simulink model "Shaddad_BMS"  (R2026b)
undefined symbols (not defined in the file): CAN, FD, P, Ts
libraries: simulink x39, stm32blockslib x12, BatteryProtection x7, dspstat3 x7, BatteryEstimators x4, BatteryCurrentManagement x3, eeGeneralControl x2, BatteryBalancing x1, BatterySoeEstimators x1, BatteryPowerEstimators x1, BatteryThermalManagement x1, svdutilitieslib x1
(part 1 of 2)
settings Model: Creator=aomar  LastModifiedBy=aomar

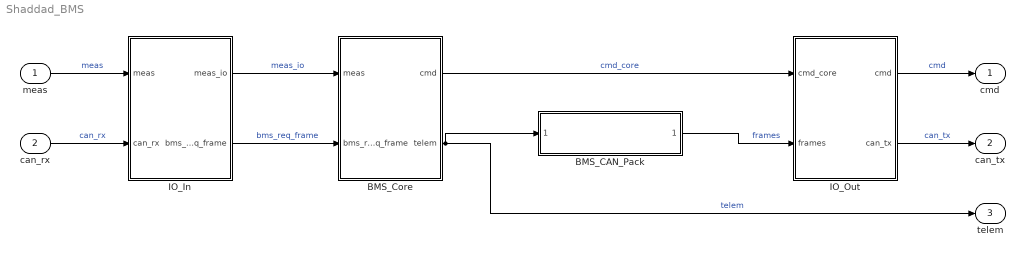
== system Shaddad_BMS ==
  meas : Inport  OutDataTypeStr=Bus: Bus_BMS_Meas  SampleTime=Ts.bms_fast  BusOutputAsStruct=on
  can_rx : Inport  Port=2  OutDataTypeStr=Bus: Bus_Can1_McuSlow  SampleTime=Ts.can_slow  BusOutputAsStruct=on
  BMS_CAN_Pack : Subsystem  ReferencedSubsystem=bms_can_pack
  BMS_Core : Subsystem  TreatAsAtomicUnit=on
  IO_In : Subsystem  Variant=on
  IO_Out : Subsystem  Variant=on
  cmd : Outport  OutDataTypeStr=Bus: Bus_BMS_Cmd  SampleTime=Ts.bms_fast  BusOutputAsStruct=on
  can_tx : Outport  Port=2  OutDataTypeStr=Bus: Bus_Can1_Bms  SampleTime=Ts.hk  BusOutputAsStruct=on
  telem : Outport  Port=3  OutDataTypeStr=Bus: Bus_BMS_Telemetry  SampleTime=Ts.hk  BusOutputAsStruct=on
  wires:
  meas/1 -> IO_In/1(meas)  "meas"
  can_rx/1 -> IO_In/2(can_rx)  "can_rx"
  IO_In/1(meas_io) -> BMS_Core/1(meas)  "meas_io"
  IO_In/2(bms_req_frame) -> BMS_Core/2(bms_req_frame)  "bms_req_frame"
  BMS_Core/1(cmd) -> IO_Out/1(cmd_core)  "cmd_core"
  BMS_Core/2(telem) -> telem/1, BMS_CAN_Pack/1  "telem"
  BMS_CAN_Pack/1 -> IO_Out/2(frames)  "frames"
  IO_Out/1(cmd) -> cmd/1  "cmd"
  IO_Out/2(can_tx) -> can_tx/1  "can_tx"

== system Shaddad_BMS/BMS_Core ==
  meas : Inport  OutDataTypeStr=Bus: Bus_BMS_Meas
  bms_req_frame : Inport  Port=2  OutDataTypeStr=Bus: Bus_CanFrame8
  BMS_REQ_Decode : Subsystem  ReferencedSubsystem=bmsreq_can_unpack
  Balancing : Subsystem  Description=Balancing (1 s): E16 Passive Cell Balancing (10 mV threshold, 3 mV hysteresis) enabled when (CHARGING or REST) and V_max > 3.40 V; E6 cell contact monitoring (gated off by P.power.bms.contact_enable).
  ChargeCtrl : Subsystem  Description=Charge control (0.1 s): E15 CC-CV on V_max (CV 3.55 V), request = min(CC-CV, I_chg_lim, 100 A) while CHARGING; E21 charge complete (V_max >= 3.545 V and I < 10 A for 60 s).
  CmdOut : Subsystem  Description=Bus_BMS_Cmd assembly; balancing gated at 10 ms ((CHARGING (K4 request) or |I| < I_rest) and V_max > 3.40 V); Unit Delay (0.01 s) = BMS output stage and the plant -> BMS -> plant loop breaker (E24).
  Estimation : Subsystem  Description=Estimation (0.1 s; capacity LS at 1 s): E7 SOC EKF x16 (variable capacity, D48; cell voltages corrected by the R0 ageing ratio R0a_* learned at current steps), E8 coulomb counting, E10 capacity (rate limit AH_rate_lim, bounds AH_bounds), E11 SOH, E12 SOE (EnergyCapacity = CellAH x 51.2 V), E9 power capability, E20 moving average of P_pack (P_avg_window samples at 1 s = 600 s), E_remaining = E_cap x max(SOC_pack - 0.10, 0), Runtime = 3600 E_remaining / max(P_avg, 200 W).
  FaultWord : Subsystem  Description=Fault_Word = latched protection bits | b6 PRECHARGE_FAIL | b7 K1_WELD | b16 SAFETY_OPEN | b20 MCU_CMD_TIMEOUT (b17-19 LV: no rail measurement at the BMS); Warning_Word b0-b7; Fault_Level 3/2/1/0 from P.power.bms.fault masks.
  Limits : Subsystem  Description=Current limits (0.01 s): E13 / E14 (MinMax inputs, temperature tables, voltage headroom), E22 SOC taper on SOC_min, peak / charge maxima. Outputs are magnitudes (A).
  Meas : Subsystem  Description=Measurement conditioning (0.01 s): min/max with index (dspstat3), mean, [min;max] pairs, I_lib = -I_pack (batt_sl_lib + = charge), P_pack.
  ModeManager : Subsystem  Description=Mode manager (0.01 s): MATLAB Function BMS_ModeManager (spec 4.1 transition table, enum BmsContactorState, after() tick counters, P.power.bms.chart), Safety_OK input = meas.Safety_HV_OK (stop-category-1 coil supply), MCU command timeout (BMS_REQ alive frozen 0.5 s -> HV_Enable_Req false, Fault_Word b20), Fault_Reset_Req rising edge for the protection latch.
  Protection : Subsystem  Description=Protection (0.01 s): E1 critical / E2 warning voltage monitoring, E3 overcurrent, E4 temperature, E5 fault qualification (fuses, charger OVP), E6 gate; fault bits latched until a Fault_Reset_Req rising edge with the symptom gone (library DisqualTime 0 would never clear, so P.power.bms.disqual is used).
  RT_req : RateTransition  OutPortSampleTime=Ts.bms_fast
  RT_req_valid : RateTransition  OutPortSampleTime=Ts.bms_fast
  Telemetry : Subsystem  Description=Telemetry (0.1 s): Bus_BMS_Telemetry with AliveCounter (+1 per 0.1 s), fault / warning words, contactor state, CVL / DVL.
  Thermal : Subsystem  Description=Fan control (0.1 s): E17 Battery Coolant Control ON-OFF 40 / 35 C on [T_min; T_max], AND T_max > T_amb - 1 K, OR T_max > 50 C.
  cmd : Outport  OutDataTypeStr=Bus: Bus_BMS_Cmd
  telem : Outport  Port=2  OutDataTypeStr=Bus: Bus_BMS_Telemetry
  wires:
  meas/1 -> Meas/1(meas)  "meas"
  bms_req_frame/1 -> BMS_REQ_Decode/1  "bms_req_frame"
  Meas/1(m) -> Limits/1(m), Thermal/1(m), ChargeCtrl/1(m), Protection/1(m), Telemetry/1(m), FaultWord/1(m), Balancing/1(m), Estimation/1(m), CmdOut/1(m), ModeManager/1(m)  "m"
  BMS_REQ_Decode/1 -> RT_req/1  "bms_req"
  BMS_REQ_Decode/2 -> RT_req_valid/1  "bms_req_valid"
  RT_req/1 -> ModeManager/2(req)  "req"
  RT_req_valid/1 -> ModeManager/3(req_valid)  "req_valid"
  Estimation/1(est) -> Limits/2(est), Telemetry/3(est), FaultWord/4(est)  "est"
  Thermal/1(Fan_Cmd) -> CmdOut/4(Fan_Cmd), FaultWord/6(Fan_Cmd), Telemetry/7(Fan_Cmd)  "Fan_Cmd"
  ModeManager/1(mode) -> CmdOut/2(mode), ChargeCtrl/2(mode), Balancing/2(mode), FaultWord/3(mode), Protection/2(mode), Telemetry/2(mode)  "mode"
  Limits/1(I_dis_lim) -> Protection/4(I_dis_lim), Telemetry/5(I_dis_lim)  "I_dis_lim"
  Limits/2(I_chg_lim) -> Protection/3(I_chg_lim), ChargeCtrl/3(I_chg_lim), Telemetry/6(I_chg_lim)  "I_chg_lim"
  Limits/3(derate) -> FaultWord/5(derate)  "derate"
  Balancing/1(Bal_Cmd) -> CmdOut/3(Bal_Cmd)  "Bal_Cmd"
  Balancing/2(Balancing_Active) -> Telemetry/9(Balancing_Active)  "Balancing_Active"
  Balancing/3(contact_err) -> Protection/5(contact_err)  "contact_err"
  ChargeCtrl/1(I_req) -> CmdOut/5(I_req)  "I_req"
  ChargeCtrl/2(ChargeComplete) -> ModeManager/5(ChargeComplete)  "ChargeComplete"
  CmdOut/1(cmd) -> cmd/1  "cmd"
  CmdOut/2(Bal_Cmd_out) -> Telemetry/8(Bal_Cmd)  "Bal_Cmd_out"
  Protection/1(prot) -> FaultWord/2(prot), ModeManager/4(prot)  "prot"
  FaultWord/1(fw) -> Telemetry/4(fw)  "fw"
  Telemetry/1(telem) -> telem/1  "telem"

== system Shaddad_BMS/IO_In ==
  note: 1) Add Subsystem or Model blocks as valid variant choices.
      | 2) You cannot connect blocks at this level. At simulation, connectivity is automatically
      | determined, based on the active variant and port name matching.
  meas : Inport
  can_rx : Inport  Port=2
  HW : Subsystem  Description=HW IO_In (VC_TARGET == 1): SPI AFE + afe_decode (block-based register decode), ADC1 6 channels, GPIO aux contacts (Digital Port Read GPIOC[4:11], one boolean per pin -> Demux), FDCAN1 read of 0x3D0 (Data [64x1] -> bytes 1:8, Length, Id; valid = Id == BMS_REQ). Peripheral settings / pin maps are configured by T17 (CubeMX, build_targets('peripherals')).  VariantControl=VC_TARGET == 1
  SIM : Subsystem  VariantControl=VC_TARGET == 0
  meas_io : Outport
  bms_req_frame : Outport  Port=2

== system Shaddad_BMS/IO_Out ==
  note: 1) Add Subsystem or Model blocks as valid variant choices.
      | 2) You cannot connect blocks at this level. At simulation, connectivity is automatically
      | determined, based on the active variant and port name matching.
  cmd_core : Inport
  frames : Inport  Port=2
  HW : Subsystem  Description=HW IO_Out (VC_TARGET == 1): contactor / charger / balancing GPIO, FDCAN1 raw-data transmit of the 7 BMS frames (inputs Data, Length, Id; Digital Port Write GPIOB[4 5 6 7 10] = K1 K2 K4 CHARGER_EN BAL_EN = OR(Bal_Cmd); pin maps from shaddad_g474.ioc, T17). Root outputs keep the SIM buses.  VariantControl=VC_TARGET == 1
  SIM : Subsystem  VariantControl=VC_TARGET == 0
  cmd : Outport
  can_tx : Outport  Port=2

== system Shaddad_BMS/BMS_Core/Balancing ==
  m_V_cell : Inport  PortName=m  Element=V_cell
  m_V_max : Inport  PortName=m  Element=V_max
  m_I_dis : Inport  PortName=m  Element=I_dis
  mode_Charging_Active : Inport  Port=2  PortName=mode  Element=Charging_Active
  Bal_enable : Logic  AllPortsSameDT=off  OutDataTypeStr=boolean
  Chg_or_rest : Logic  Operator=OR  AllPortsSameDT=off  OutDataTypeStr=boolean
  E16_Passive_balancing : BatteryBalancing/Passive Cell Balancing  Threshold=single(P.power.bms.bal.Threshold)  HysteresisBand=single(P.power.bms.bal.Hyst)  Td_on=P.power.bms.bal.Td_on  Td_off=P.power.bms.bal.Td_off  Ts=Ts.bms_bal  dataType=boolean
      settings: LibrarySourceBlock=batt_sl_lib/Cell Balancing/Passive Cell Balancing
  E6_Cell_contact : BatteryProtection/Battery Cell Contact Monitoring  Td=10  VoltageChangeDetectionThreshold=single(5e-4)  VoltageChangePar=single(0.02)  CumulativeErrorThreshold=single(1e-4)  QualTime=20  DisqualTime=0  Ts=Ts.bms_bal  DataType=single
      settings: LibrarySourceBlock=|
      | batt_sl_lib/Protection/Battery Cell Contact
      | Monitoring
  E6_any : Logic  Operator=OR  Inputs=1  AllPortsSameDT=off  OutDataTypeStr=boolean
  E6_symptom : Terminator
  I_abs : Abs  SaturateOnIntegerOverflow=off
  RT_I_dis : RateTransition  OutPortSampleTime=Ts.bms_bal
  RT_V_cell : RateTransition  OutPortSampleTime=Ts.bms_bal
  RT_V_max : RateTransition  OutPortSampleTime=Ts.bms_bal
  RT_active : RateTransition  OutPortSampleTime=Ts.bms_bal
  RT_contact : RateTransition  OutPortSampleTime=Ts.bms_fast
  Rest : simulink/Logic and Bit Operations/Compare To Constant  relop=<  const=single(P.power.bms.I_rest)  OutDataTypeStr=boolean
  Top : simulink/Logic and Bit Operations/Compare To Constant  relop=>  const=single(P.power.bms.V_bal_enable)  OutDataTypeStr=boolean
  Bal_Cmd : Outport
  Balancing_Active : Outport  Port=2
  contact_err : Outport  Port=3
  wires:
  m_I_dis/1 -> RT_I_dis/1  "I_dis"
  m_V_cell/1 -> RT_V_cell/1  "V_cell"
  RT_I_dis/1 -> I_abs/1  "RT_I_dis"
  RT_V_cell/1 -> E16_Passive_balancing/1, E6_Cell_contact/1  "RT_V_cell"
  I_abs/1 -> Rest/1  "I_abs"
  E6_Cell_contact/1 -> E6_any/1  "E6_Cell_contact_1"
  E6_Cell_contact/2 -> E6_symptom/1  "E6_Cell_contact_2"
  mode_Charging_Active/1 -> RT_active/1  "Charging_Active"
  m_V_max/1 -> RT_V_max/1  "V_max"
  Rest/1 -> Chg_or_rest/2  "Rest"
  RT_active/1 -> Chg_or_rest/1  "RT_active"
  RT_V_max/1 -> Top/1  "RT_V_max"
  Chg_or_rest/1 -> Bal_enable/1  "Chg_or_rest"
  Top/1 -> Bal_enable/2  "Top"
  Bal_enable/1 -> E16_Passive_balancing/2  "bal_enable"
  E6_any/1 -> RT_contact/1  "E6_any"
  RT_contact/1 -> contact_err/1  "contact_err"
  E16_Passive_balancing/1 -> Bal_Cmd/1  "Bal_Cmd"
  E16_Passive_balancing/2 -> Balancing_Active/1  "Balancing_Active"

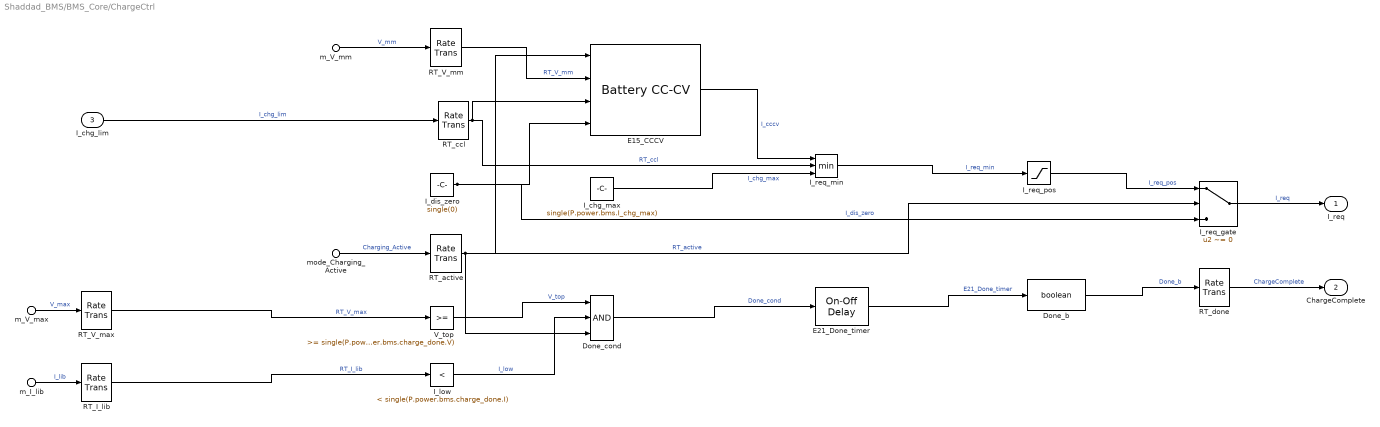
== system Shaddad_BMS/BMS_Core/ChargeCtrl ==
  m_V_mm : Inport  PortName=m  Element=V_mm
  m_V_max : Inport  PortName=m  Element=V_max
  m_I_lib : Inport  PortName=m  Element=I_lib
  mode_Charging_Active : Inport  Port=2  PortName=mode  Element=Charging_Active
  I_chg_lim : Inport  Port=3
  Done_b : DataTypeConversion  OutDataTypeStr=boolean  SaturateOnIntegerOverflow=off  RndMeth=Floor
  Done_cond : Logic  Inputs=3  AllPortsSameDT=off  OutDataTypeStr=boolean
  E15_CCCV : BatteryCurrentManagement/Battery CC-CV  MinMaxFlag=on  MaxCellVoltage=single(P.power.bms.V_cv)  Kp=single(P.power.bms.cccv.Kp)  Ki=single(P.power.bms.cccv.Ki)  Kaw=single(P.power.bms.cccv.Kaw)  Kt=single(P.power.bms.cccv.Kt)  Ts=Ts.bms_slow
      settings: LibrarySourceBlock=batt_sl_lib/Current Management/Battery CC-CV
  E21_Done_timer : eeGeneralControl/On-Off Delay  LabelModeActiveChoice=Discrete  Td_on=P.power.bms.charge_done.t  Td_off=0  IC=0  Ts=Ts.bms_slow
      settings: LibrarySourceBlock=ee_sl_lib/General Control/On-Off Delay
  I_chg_max : Constant  Value=single(P.power.bms.I_chg_max)  OutDataTypeStr=single  SampleTime=Ts.bms_slow
  I_dis_zero : Constant  Value=single(0)  OutDataTypeStr=single  SampleTime=Ts.bms_slow
  I_low : simulink/Logic and Bit Operations/Compare To Constant  relop=<  const=single(P.power.bms.charge_done.I)  OutDataTypeStr=boolean
  I_req_gate : Switch  Criteria=u2 ~= 0  SaturateOnIntegerOverflow=off  InputSameDT=off
  I_req_min : MinMax  Inputs=3
  I_req_pos : Saturate  UpperLimit=inf  LowerLimit=single(0)
  RT_I_lib : RateTransition  OutPortSampleTime=Ts.bms_slow
  RT_V_max : RateTransition  OutPortSampleTime=Ts.bms_slow
  RT_V_mm : RateTransition  OutPortSampleTime=Ts.bms_slow
  RT_active : RateTransition  OutPortSampleTime=Ts.bms_slow
  RT_ccl : RateTransition  OutPortSampleTime=Ts.bms_slow
  RT_done : RateTransition  OutPortSampleTime=Ts.bms_fast
  V_top : simulink/Logic and Bit Operations/Compare To Constant  relop=>=  const=single(P.power.bms.charge_done.V)  OutDataTypeStr=boolean
  I_req : Outport
  ChargeComplete : Outport  Port=2
  wires:
  m_V_max/1 -> RT_V_max/1  "V_max"
  m_I_lib/1 -> RT_I_lib/1  "I_lib"
  I_chg_lim/1 -> RT_ccl/1  "I_chg_lim"
  RT_V_max/1 -> V_top/1  "RT_V_max"
  RT_I_lib/1 -> I_low/1  "RT_I_lib"
  m_V_mm/1 -> RT_V_mm/1  "V_mm"
  mode_Charging_Active/1 -> RT_active/1  "Charging_Active"
  I_dis_zero/1 -> E15_CCCV/4, I_req_gate/3  "I_dis_zero"
  V_top/1 -> Done_cond/1  "V_top"
  I_low/1 -> Done_cond/2  "I_low"
  RT_V_mm/1 -> E15_CCCV/2  "RT_V_mm"
  RT_active/1 -> E15_CCCV/1, Done_cond/3, I_req_gate/2  "RT_active"
  RT_ccl/1 -> I_req_min/2, E15_CCCV/3  "RT_ccl"
  I_chg_max/1 -> I_req_min/3  "I_chg_max"
  Done_cond/1 -> E21_Done_timer/1  "Done_cond"
  E15_CCCV/1 -> I_req_min/1  "I_cccv"
  I_req_min/1 -> I_req_pos/1  "I_req_min"
  E21_Done_timer/1 -> Done_b/1  "E21_Done_timer"
  I_req_pos/1 -> I_req_gate/1  "I_req_pos"
  Done_b/1 -> RT_done/1  "Done_b"
  RT_done/1 -> ChargeComplete/1  "ChargeComplete"
  I_req_gate/1 -> I_req/1  "I_req"

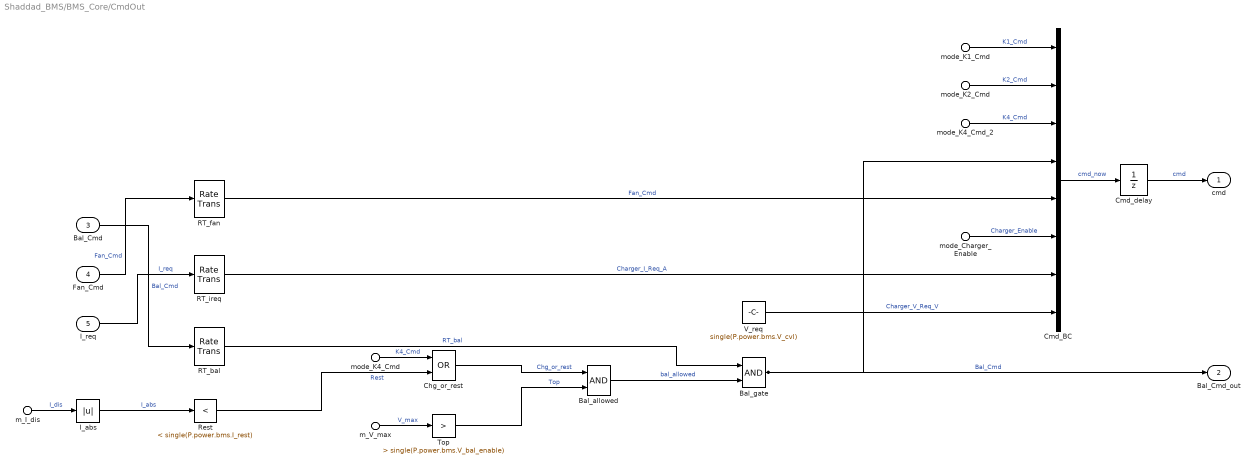
== system Shaddad_BMS/BMS_Core/CmdOut ==
  m_I_dis : Inport  PortName=m  Element=I_dis
  m_V_max : Inport  PortName=m  Element=V_max
  mode_K4_Cmd : Inport  Port=2  PortName=mode  Element=K4_Cmd
  mode_K4_Cmd_2 : Inport  Port=2  PortName=mode  Element=K4_Cmd
  mode_K1_Cmd : Inport  Port=2  PortName=mode  Element=K1_Cmd
  mode_K2_Cmd : Inport  Port=2  PortName=mode  Element=K2_Cmd
  mode_Charger_Enable : Inport  Port=2  PortName=mode  Element=Charger_Enable
  Bal_Cmd : Inport  Port=3
  Fan_Cmd : Inport  Port=4
  I_req : Inport  Port=5
  Bal_allowed : Logic  AllPortsSameDT=off  OutDataTypeStr=boolean
  Bal_gate : Logic  AllPortsSameDT=off  OutDataTypeStr=boolean
  Chg_or_rest : Logic  Operator=OR  AllPortsSameDT=off  OutDataTypeStr=boolean
  Cmd_BC : BusCreator  Inputs=8  OutDataTypeStr=Bus: Bus_BMS_Cmd  NonVirtualBus=on
      settings: InheritFromInputs=off
  Cmd_delay : UnitDelay  InitialCondition=P.ic.Bus_BMS_Cmd  SampleTime=Ts.bms_fast
  I_abs : Abs  SaturateOnIntegerOverflow=off
  RT_bal : RateTransition  OutPortSampleTime=Ts.bms_fast
  RT_fan : RateTransition  OutPortSampleTime=Ts.bms_fast
  RT_ireq : RateTransition  OutPortSampleTime=Ts.bms_fast
  Rest : simulink/Logic and Bit Operations/Compare To Constant  relop=<  const=single(P.power.bms.I_rest)  OutDataTypeStr=boolean
  Top : simulink/Logic and Bit Operations/Compare To Constant  relop=>  const=single(P.power.bms.V_bal_enable)  OutDataTypeStr=boolean
  V_req : Constant  Value=single(P.power.bms.V_cvl)  OutDataTypeStr=single  SampleTime=Ts.bms_fast
  cmd : Outport
  Bal_Cmd_out : Outport  Port=2
  wires:
  m_I_dis/1 -> I_abs/1  "I_dis"
  Bal_Cmd/1 -> RT_bal/1  "Bal_Cmd"
  Fan_Cmd/1 -> RT_fan/1  "Fan_Cmd"
  I_req/1 -> RT_ireq/1  "I_req"
  I_abs/1 -> Rest/1  "I_abs"
  Rest/1 -> Chg_or_rest/2  "Rest"
  RT_fan/1 -> Cmd_BC/5  "Fan_Cmd"
  RT_ireq/1 -> Cmd_BC/7  "Charger_I_Req_A"
  RT_bal/1 -> Bal_gate/1  "RT_bal"
  mode_K4_Cmd/1 -> Chg_or_rest/1  "K4_Cmd"
  m_V_max/1 -> Top/1  "V_max"
  Chg_or_rest/1 -> Bal_allowed/1  "Chg_or_rest"
  Top/1 -> Bal_allowed/2  "Top"
  Bal_allowed/1 -> Bal_gate/2  "bal_allowed"
  V_req/1 -> Cmd_BC/8  "Charger_V_Req_V"
  Bal_gate/1 -> Cmd_BC/4, Bal_Cmd_out/1  "Bal_Cmd"
  mode_K1_Cmd/1 -> Cmd_BC/1  "K1_Cmd"
  mode_K2_Cmd/1 -> Cmd_BC/2  "K2_Cmd"
  mode_K4_Cmd_2/1 -> Cmd_BC/3  "K4_Cmd"
  mode_Charger_Enable/1 -> Cmd_BC/6  "Charger_Enable"
  Cmd_BC/1 -> Cmd_delay/1  "cmd_now"
  Cmd_delay/1 -> cmd/1  "cmd"

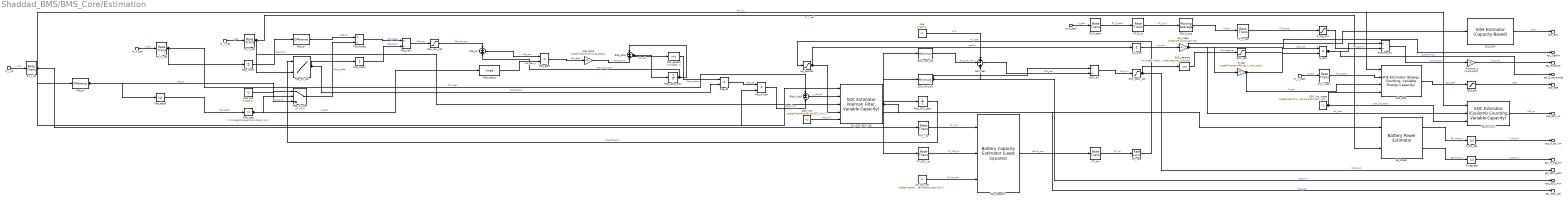
== system Shaddad_BMS/BMS_Core/Estimation ==
  m_I_lib : Inport  PortName=m  Element=I_lib
  m_V_cell : Inport  PortName=m  Element=V_cell
  m_T_cell : Inport  PortName=m  Element=T_cell
  m_V_pack : Inport  PortName=m  Element=V_pack
  m_P_pack : Inport  PortName=m  Element=P_pack
  AH_bounds : Saturate  UpperLimit=single(P.power.bms.est.AH_bounds(2))  LowerLimit=single(P.power.bms.est.AH_bounds(1))
  AH_init_vec : Constant  Value=single(P.power.bms.est.AH_init*ones(P.power.pack.Ns,1))  OutDataTypeStr=single  SampleTime=Ts.bms_bal
  AH_mean : Gain  Gain=single(1/P.power.pack.Ns)
  AH_rate : RateLimiter  RisingSlewLimit=single(P.power.bms.est.AH_rate_lim)  FallingSlewLimit=single(-P.power.bms.est.AH_rate_lim)  SampleTimeMode=inherited  InitialCondition=single(P.power.bms.est.AH_init)
  AH_sum : Sum  Inputs=+
  E10_Capacity : BatteryEstimators/Battery Capacity Estimator (Least Squares)  CurrentInputPartition=off  lsAlgorithm=Ordinary least squares  SocChangeThreshold=single(P.power.bms.cap_est.SocChangeThreshold)  gamma=single(P.power.bms.cap_est.gamma)  VarianceX=2e-4  VarianceY=5e-7  k=10  Ts=P.power.bms.cap_est.Ts  DataType=single
      settings: LibrarySourceBlock=|
      | batt_sl_lib/Estimators/Battery Capacity Estimator
      | (Least Squares)
  E11_SOH : BatteryEstimators/SOH Estimator (Capacity-Based)  AH_new=single(P.power.bms.soh.AH_new)  AH_eol=single(P.power.bms.soh.AH_eol)  DataType=single
      settings: LibrarySourceBlock=batt_sl_lib/Estimators/SOH Estimator (Capacity-Based)
  E12_SOE : BatterySoeEstimators/SOE Estimator (Energy Counting, Variable Energy Capacity)  CurrentInputPartition=off  Ts=Ts.bms_slow  DataType=single
      settings: LibrarySourceBlock=|
      | batt_sl_lib/Estimators/SOE Estimator (Energy Counting,
      | Variable Energy Capacity)
  E20_P_avg : dspstat3/Moving Average  Method=Sliding window  ForgettingFactorPort=off  SpecifyWindowLength=on  WindowLengthSource=Property  MaxWindowLength=20  WindowLength=P.power.bms.P_avg_window  OverlapLength=P.power.bms.P_avg_window - 1  AllowArbitraryInputLength=off  ForgettingFactor=0.9  SimulateUsing=Interpreted execution
  E7_SOC_EKF_x16 : BatteryEstimators/SOC Estimator (Kalman Filter, Variable Capacity)  CurrentInputPartition=off  filterType=Extended Kalman filter  alpha=1  beta=2  kappa=0  Q=single(P.power.bms.ekf.Q)  Q_2RC=|  R=single(P.power.bms.ekf.R)  P0=single(P.power.bms.ekf.P0)  P0_2RC=[1e-5 0 0; 0 1 0;0 0 1]  Ts=Ts.bms_slow  chargeDynamics=One time-constant dynamics  SOC_vec=single(P.power.group.SOC_vec)  T_vec=single(P.power.group.T_vec)  R0_mat=single(P.power.group.R0_mat)  R1_mat=single(P.power.group.R1_mat)  tau1_mat=single(P.power.group.tau1_mat)  R2_mat=[.0109, .0029, .0013; .0069, .0024, .0012; .0047, .0026, .0013; .0034, .0016, .001; .0033, .0023, .0014; .0033, .0018, .0011; .0028, .0017, .0011]  tau2_mat=[20, 36, 39; 31, 45, 39; 109, 105, 61; 36, 29, 26; 59, 77, 67; 40, 33, 29; 25, 39, 33]  V0_mat=single(P.power.group.V0_mat)  DataType=single
      | [1e-6 0 0;
      | 0 1e-6 0;0 0 1e-6]
      settings: LibrarySourceBlock=|
      | batt_sl_lib/Estimators/SOC Estimator
      | (Kalman Filter, Variable Capacity)
  E8_SOC_CC : BatteryEstimators/SOC Estimator (Coulomb Counting, Variable Capacity)  CurrentInputPartition=off  Ts=Ts.bms_slow  DataType=single
      settings: LibrarySourceBlock=|
      | batt_sl_lib/Estimators/SOC Estimator
      | (Coulomb Counting, Variable Capacity)
  E9_Power : BatteryPowerEstimators/Battery Power Estimator  SOC_vec=single(P.power.group.SOC_vec)  T_vec=single(P.power.group.T_vec)  V0_mat=single(P.power.group.V0_mat)  R0ChargingTimeHorizon=single(P.power.bms.pwr_est.R_10s)  R0DischargingTimeHorizon=single(P.power.bms.pwr_est.R_10s)  AH=single(P.power.group.AH)  Ns=P.power.pack.Ns  Np=1  ChargingEfficiency=single(P.power.bms.pwr_est.ChargingEfficiency)  vmin=single(P.power.bms.pwr_est.vmin)  vmax=single(P.power.bms.pwr_est.vmax)  SOCmin=single(P.power.bms.pwr_est.SOCmin)  SOCmax=single(P.power.bms.pwr_est.SOCmax)  imin=single(P.power.bms.pwr_est.imin)  imax=single(P.power.bms.pwr_est.imax)  Pmin=single(P.power.bms.pwr_est.Pmin)  Pmax=single(P.power.bms.pwr_est.Pmax)  TimeHorizon=single(P.power.bms.pwr_est.TimeHorizon)  DataType=single
      settings: LibrarySourceBlock=batt_sl_lib/Estimators/Battery Power Estimator
  E_cap : Gain  Gain=single(P.power.bms.est.V_nom_pack)
  E_rem : Product
  P_avg_min : Saturate  UpperLimit=inf  LowerLimit=single(P.power.bms.runtime_P_min)
  P_chg_abs : Abs  SaturateOnIntegerOverflow=off
  P_dis_abs : Abs  SaturateOnIntegerOverflow=off
  R0a_R0_tab : Lookup_n-D  BreakpointsForDimension1=single(P.power.group.SOC_vec)  BreakpointsForDimension2=single(P.power.group.T_vec)  BreakpointsForDimension3=[5, 7]  Table=single(P.power.group.R0_mat)  ExtrapMethod=Clip  InternalRulePriority=Speed  OutDataTypeStr=single  RndMeth=Simplest
      settings: InputPortMap=u0,u1
  R0a_Rstep : Product  Inputs=*/
  R0a_Rsum : Sum  Inputs=+
  R0a_SOC_prev : UnitDelay  InitialCondition=single(P.power.bms.est.SOC_init(:))  SampleTime=Ts.bms_slow
  R0a_V_ekf : Sum  Inputs=+-
  R0a_Vsum : Sum  Inputs=+
  R0a_absdI : Abs  SaturateOnIntegerOverflow=off
  R0a_alpha : Gain  Gain=single(P.power.bms.r0a.alpha)
  R0a_dI : simulink/Discrete/Difference  ICPrevInput=single(0)  OutMin=[]  OutMax=[]  OutDataTypeStr=single  OutputDataTypeScalingMode=single  OutDataType=fixdt(1, 16)  OutScaling=2^-10  DoSatur=off
  R0a_dI_safe : Switch  Criteria=u2 ~= 0  SaturateOnIntegerOverflow=off  InputSameDT=off
  R0a_dR : Product
  R0a_dV : simulink/Discrete/Difference  ICPrevInput=single(0)  OutMin=[]  OutMax=[]  OutDataTypeStr=single  OutputDataTypeScalingMode=single  OutDataType=fixdt(1, 16)  OutScaling=2^-10  DoSatur=off
  R0a_dVcorr : Product
  R0a_err : Sum  Inputs=+-
  R0a_excess : Bias  Bias=single(-1)  SaturateOnIntegerOverflow=off
  R0a_gate : Product
  R0a_one : Constant  Value=single(1)  OutDataTypeStr=single  SampleTime=Ts.bms_slow
  R0a_ratio : Sum
  R0a_ratio_prev : UnitDelay  InitialCondition=single(P.power.bms.r0a.ratio_init)  SampleTime=Ts.bms_slow
  R0a_raw : Product  Inputs=*/
  R0a_raw_sat : Saturate  UpperLimit=single(P.power.bms.r0a.ratio_bounds(2))  LowerLimit=single(P.power.bms.r0a.ratio_bounds(1))
  R0a_step : simulink/Logic and Bit Operations/Compare To Constant  relop=>=  const=single(P.power.bms.r0a.dI_min)  OutDataTypeStr=boolean
  R0a_step_s : DataTypeConversion  OutDataTypeStr=single  RndMeth=Nearest
  RT_AH : RateTransition  OutPortSampleTime=Ts.bms_slow
  RT_I_1s : RateTransition  OutPortSampleTime=Ts.bms_bal
  RT_I_lib : RateTransition  OutPortSampleTime=Ts.bms_slow
  RT_P_1s : RateTransition  OutPortSampleTime=Ts.bms_bal
  RT_P_avg : RateTransition  OutPortSampleTime=Ts.bms_slow
  RT_P_pack : RateTransition  OutPortSampleTime=Ts.bms_slow
  RT_SOC_1s : RateTransition  OutPortSampleTime=Ts.bms_bal
  RT_T_cell : RateTransition  OutPortSampleTime=Ts.bms_slow
  RT_V_cell : RateTransition  OutPortSampleTime=Ts.bms_slow
  RT_V_pack : RateTransition  OutPortSampleTime=Ts.bms_slow
  Runtime_div : Product  Inputs=*/
  Runtime_s : Gain  Gain=single(3600)
  SOC_den : Sum  Inputs=+-+
  SOC_div : Product  Inputs=*/
  SOC_init : Constant  Value=single(P.power.bms.est.SOC_init(:))  OutDataTypeStr=single  SampleTime=Ts.bms_slow
  SOC_init_mean : Constant  Value=single(mean(P.power.bms.est.SOC_init))  OutDataTypeStr=single  SampleTime=Ts.bms_slow
  SOC_max_blk : dspstat3/Maximum  operation=maximum  fcn=Value  indexBase=One  operateOver=Each column  Dimension=1  InputProcessing=Columns as channels (frame based)  reset=None  roiEnable=off  roiType=Rectangles  roiPortion=Entire ROI  roiOutput=Individual statistics for each ROI  roiFlag=off  roundingMode=Floor  overflowMode=off  accumDataTypeStr=Inherit: Same as product output  accumLastDataTypeStr=Inherit: Same as product output
  SOC_min_blk : dspstat3/Minimum  operation=minimum  fcn=Value  indexBase=One  operateOver=Each column  Dimension=1  InputProcessing=Columns as channels (frame based)  reset=None  roiEnable=off  roiType=Rectangles  roiPortion=Entire ROI  roiOutput=Individual statistics for each ROI  roiFlag=off  roundingMode=Floor  overflowMode=off
  SOC_pack_sat : Saturate  UpperLimit=single(1)  LowerLimit=single(0)
  SOC_reserve : Bias  Bias=single(-P.power.bms.soc_reserve_runtime)  SaturateOnIntegerOverflow=off
  SOC_use : Saturate  UpperLimit=single(1)  LowerLimit=single(0)
  SOE_sat : Saturate  UpperLimit=single(1)  LowerLimit=single(0)
  one : Constant  Value=single(1)  OutDataTypeStr=single  SampleTime=Ts.bms_slow
  est_SOC_cell : Outport  PortName=est  Element=SOC_cell
  est_CellAH : Outport  PortName=est  Element=CellAH
  est_SOC_cc : Outport  PortName=est  Element=SOC_cc
  est_SOH : Outport  PortName=est  Element=SOH
  est_SOE : Outport  PortName=est  Element=SOE
  est_SOC_pack : Outport  PortName=est  Element=SOC_pack
  est_SOC_min : Outport  PortName=est  Element=SOC_min
  est_P_dis_lim : Outport  PortName=est  Element=P_dis_lim
  est_P_chg_lim : Outport  PortName=est  Element=P_chg_lim
  est_E_remaining : Outport  PortName=est  Element=E_remaining
  est_Runtime : Outport  PortName=est  Element=Runtime
  wires:
  m_I_lib/1 -> RT_I_lib/1  "I_lib"
  RT_I_lib/1 -> RT_I_1s/1, E8_SOC_CC/1, R0a_dVcorr/2, E7_SOC_EKF_x16/1, R0a_dI/1, E12_SOE/1  "RT_I_lib"
  R0a_dI/1 -> R0a_absdI/1, R0a_dI_safe/1  "R0a_dI"
  m_V_cell/1 -> RT_V_cell/1  "V_cell"
  R0a_absdI/1 -> R0a_step/1  "R0a_absdI"
  RT_V_cell/1 -> R0a_V_ekf/1, R0a_Vsum/1  "RT_V_cell"
  m_T_cell/1 -> RT_T_cell/1  "T_cell"
  R0a_Vsum/1 -> R0a_dV/1  "R0a_Vsum"
  R0a_one/1 -> R0a_dI_safe/3  "R0a_one"
  R0a_step/1 -> R0a_step_s/1, R0a_dI_safe/2  "r0_step"
  RT_T_cell/1 -> E9_Power/2, E7_SOC_EKF_x16/3, R0a_R0_tab/2  "RT_T_cell"
  R0a_dI_safe/1 -> R0a_Rstep/2  "R0a_dI_safe"
  R0a_dV/1 -> R0a_Rstep/1  "R0a_dV"
  R0a_R0_tab/1 -> R0a_dR/2, R0a_Rsum/1  "R0a_R0_tab"
  R0a_Rstep/1 -> R0a_raw/1  "R0a_Rstep"
  R0a_Rsum/1 -> R0a_raw/2  "R0a_Rsum"
  R0a_raw/1 -> R0a_raw_sat/1  "R0a_raw"
  R0a_raw_sat/1 -> R0a_err/1  "R0a_raw_sat"
  R0a_err/1 -> R0a_gate/1  "R0a_err"
  R0a_step_s/1 -> R0a_gate/2  "R0a_step_s"
  R0a_gate/1 -> R0a_alpha/1  "R0a_gate"
  R0a_alpha/1 -> R0a_ratio/2  "R0a_alpha"
  R0a_ratio/1 -> R0a_ratio_prev/1, R0a_excess/1  "R0_ratio"
  R0a_ratio_prev/1 -> R0a_ratio/1, R0a_err/2  "R0a_ratio_prev"
  R0a_excess/1 -> R0a_dR/1  "R0a_excess"
  R0a_dR/1 -> R0a_dVcorr/1  "R0a_dR"
  R0a_dVcorr/1 -> R0a_V_ekf/2  "R0a_dVcorr"
  R0a_V_ekf/1 -> E7_SOC_EKF_x16/2  "V_cell_ekf"
  AH_bounds/1 -> E7_SOC_EKF_x16/4, AH_sum/1  "CellAH"
  SOC_init/1 -> E7_SOC_EKF_x16/5  "SOC_init"
  E7_SOC_EKF_x16/1 -> est_SOC_cell/1, SOC_max_blk/1, RT_SOC_1s/1, SOC_min_blk/1, E9_Power/1, R0a_SOC_prev/1  "SOC_cell"
  one/1 -> SOC_den/1  "one"
  AH_init_vec/1 -> E10_Capacity/3  "AH_init_vec"
  R0a_SOC_prev/1 -> R0a_R0_tab/1  "R0a_SOC_prev"
  RT_I_1s/1 -> E10_Capacity/1  "RT_I_1s"
  RT_SOC_1s/1 -> E10_Capacity/2  "RT_SOC_1s"
  SOC_max_blk/1 -> SOC_den/2  "SOC_max_blk"
  SOC_min_blk/1 -> est_SOC_min/1, SOC_den/3, SOC_div/1  "SOC_min"
  SOC_den/1 -> SOC_div/2  "SOC_den"
  E10_Capacity/1 -> RT_AH/1  "CellAH_raw"
  m_P_pack/1 -> RT_P_pack/1  "P_pack"
  SOC_div/1 -> SOC_pack_sat/1  "SOC_div"
  RT_P_pack/1 -> RT_P_1s/1  "RT_P_pack"
  RT_AH/1 -> AH_rate/1  "RT_AH"
  AH_sum/1 -> AH_mean/1  "AH_sum"
  SOC_pack_sat/1 -> est_SOC_pack/1, SOC_reserve/1  "SOC_pack"
  AH_rate/1 -> AH_bounds/1  "AH_rate"
  RT_P_1s/1 -> E20_P_avg/1  "RT_P_1s"
  AH_mean/1 -> E8_SOC_CC/2, E_cap/1, E11_SOH/1, est_CellAH/1  "AH_pack"
  SOC_reserve/1 -> SOC_use/1  "SOC_reserve"
  E20_P_avg/1 -> RT_P_avg/1  "P_avg"
  SOC_use/1 -> E_rem/1  "SOC_use"
  E_cap/1 -> E_rem/2, E12_SOE/3  "E_cap"
  RT_P_avg/1 -> P_avg_min/1  "RT_P_avg"
  m_V_pack/1 -> RT_V_pack/1  "V_pack"
  P_avg_min/1 -> Runtime_div/2  "P_avg_min"
  E_rem/1 -> est_E_remaining/1, Runtime_div/1  "E_remaining"
  SOC_init_mean/1 -> E8_SOC_CC/3, E12_SOE/4  "SOC_init_mean"
  RT_V_pack/1 -> E12_SOE/2  "RT_V_pack"
  Runtime_div/1 -> Runtime_s/1  "Runtime_div"
  E12_SOE/1 -> SOE_sat/1  "E12_SOE"
  E9_Power/1 -> P_dis_abs/1  "E9_Power_1"
  E9_Power/2 -> P_chg_abs/1  "E9_Power_2"
  Runtime_s/1 -> est_Runtime/1  "Runtime"
  SOE_sat/1 -> est_SOE/1  "SOE"
  P_dis_abs/1 -> est_P_dis_lim/1  "P_dis_lim"
  P_chg_abs/1 -> est_P_chg_lim/1  "P_chg_lim"
  E8_SOC_CC/1 -> est_SOC_cc/1  "SOC_cc"
  E11_SOH/1 -> est_SOH/1  "SOH"

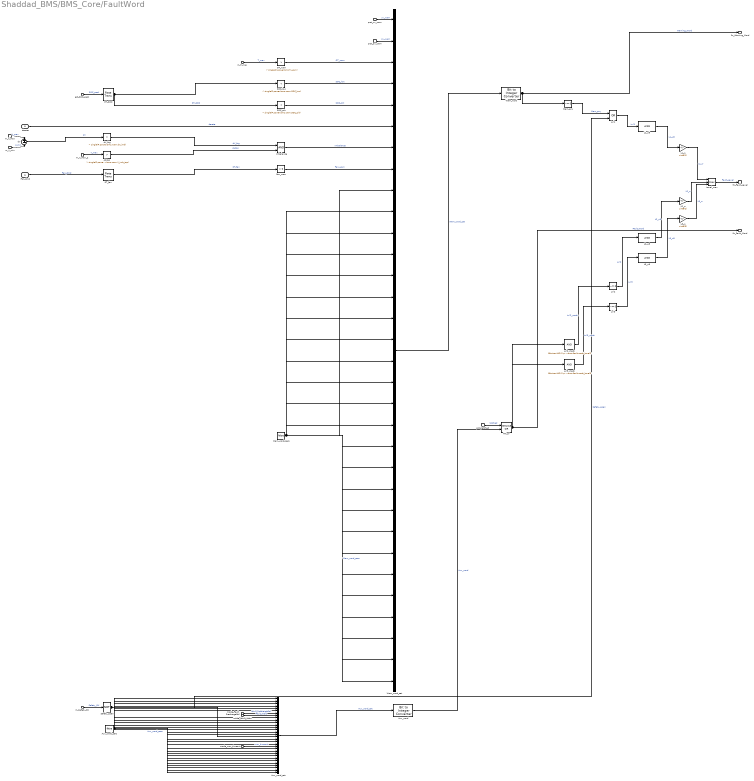
== system Shaddad_BMS/BMS_Core/FaultWord ==
  m_Safety_OK : Inport  PortName=m  Element=Safety_OK
  m_T_max : Inport  PortName=m  Element=T_max
  m_V_max : Inport  PortName=m  Element=V_max
  m_V_max_2 : Inport  PortName=m  Element=V_max
  m_V_min : Inport  PortName=m  Element=V_min
  prot_latched : Inport  Port=2  PortName=prot  Element=latched
  prot_uv_warn : Inport  Port=2  PortName=prot  Element=uv_warn
  prot_ov_warn : Inport  Port=2  PortName=prot  Element=ov_warn
  mode_Fault_PrechargeFail : Inport  Port=3  PortName=mode  Element=Fault_PrechargeFail
  mode_Fault_Weld : Inport  Port=3  PortName=mode  Element=Fault_Weld
  mode_mcu_timeout : Inport  Port=3  PortName=mode  Element=mcu_timeout
  est_SOC_pack : Inport  Port=4  PortName=est  Element=SOC_pack
  derate : Inport  Port=5
  Fan_Cmd : Inport  Port=6
  At_top : simulink/Logic and Bit Operations/Compare To Constant  relop=>  const=single(P.power.bms.warn.V_imb_top)  OutDataTypeStr=boolean
  Aux_word : simulink/Logic and Bit Operations/Bit to Integer Converter  nbits=32  bitOrder=LSB first  signedOutputValues=Unsigned  outDtype=uint32  outDtypeSigned=Inherit via internal rule
      settings: LibrarySourceBlock=|
      | commutil2/Bit to Integer
      | Converter
  Aux_word_cat : Concatenate  NumInputs=32
  Aux_word_zero : Constant  Value=false  OutDataTypeStr=boolean  SampleTime=Ts.bms_fast
  FW_or : simulink/Logic and Bit Operations/Bitwise Operator  logicop=OR  UseBitMask=off  NumInputPorts=2  BitMask=bin2dec('11011001')  BitMaskRealWorld=Stored Integer
  Fan_warn : simulink/Logic and Bit Operations/Compare To Zero  relop=>  OutDataTypeStr=boolean
  Imbalance : Logic  AllPortsSameDT=off  OutDataTypeStr=boolean
  L1_u8 : DataTypeConversion  OutDataTypeStr=uint8  RndMeth=Nearest
  L1_w : Gain  Gain=uint8(1)  ParamDataTypeStr=uint8  OutDataTypeStr=uint8
  L2_u8 : DataTypeConversion  OutDataTypeStr=uint8  RndMeth=Nearest
  L2_w : Gain  Gain=uint8(2)  ParamDataTypeStr=uint8  OutDataTypeStr=uint8
  L3_u8 : DataTypeConversion  OutDataTypeStr=uint8  RndMeth=Nearest
  L3_w : Gain  Gain=uint8(3)  ParamDataTypeStr=uint8  OutDataTypeStr=uint8
  Level_max : MinMax  Function=max  Inputs=3
  Lvl1 : Logic  Operator=OR  AllPortsSameDT=off  OutDataTypeStr=boolean
  Lvl2 : simulink/Logic and Bit Operations/Compare To Zero  relop=~=  OutDataTypeStr=boolean
  Lvl2_mask : simulink/Logic and Bit Operations/Bitwise Operator  logicop=AND  UseBitMask=on  BitMask=P.power.bms.fault.mask_level2  BitMaskRealWorld=Stored Integer
  Lvl3 : simulink/Logic and Bit Operations/Compare To Zero  relop=~=  OutDataTypeStr=boolean
  Lvl3_mask : simulink/Logic and Bit Operations/Bitwise Operator  logicop=AND  UseBitMask=on  BitMask=P.power.bms.fault.mask_level3  BitMaskRealWorld=Stored Integer
  OT_warn : simulink/Logic and Bit Operations/Compare To Constant  relop=>  const=single(P.power.bms.T_warn)  OutDataTypeStr=boolean
  RT_SOC : RateTransition  InitialCondition=single(min(P.power.bms.est.SOC_init))  OutPortSampleTime=Ts.bms_fast
  RT_fan : RateTransition  OutPortSampleTime=Ts.bms_fast
  SOC_crit : simulink/Logic and Bit Operations/Compare To Constant  relop=<  const=single(P.power.bms.warn.SOC_crit)  OutDataTypeStr=boolean
  SOC_low : simulink/Logic and Bit Operations/Compare To Constant  relop=<  const=single(P.power.bms.warn.SOC_low)  OutDataTypeStr=boolean
  Safety_open : Logic  Operator=NOT  AllPortsSameDT=off  OutDataTypeStr=boolean
  Warn_any : simulink/Logic and Bit Operations/Compare To Zero  relop=~=  OutDataTypeStr=boolean
  Warn_word : simulink/Logic and Bit Operations/Bit to Integer Converter  nbits=32  bitOrder=LSB first  signedOutputValues=Unsigned  outDtype=uint32  outDtypeSigned=Inherit via internal rule
      settings: LibrarySourceBlock=|
      | commutil2/Bit to Integer
      | Converter
  Warn_word_cat : Concatenate  NumInputs=32
  Warn_word_zero : Constant  Value=false  OutDataTypeStr=boolean  SampleTime=Ts.bms_fast
  dV : Sum  Inputs=+-
  dV_big : simulink/Logic and Bit Operations/Compare To Constant  relop=>  const=single(P.power.bms.warn.dV_imb)  OutDataTypeStr=boolean
  fw_Fault_Word : Outport  PortName=fw  Element=Fault_Word
  fw_Warning_Word : Outport  PortName=fw  Element=Warning_Word
  fw_Fault_Level : Outport  PortName=fw  Element=Fault_Level
  wires:
  m_V_max/1 -> dV/1  "V_max"
  m_V_min/1 -> dV/2  "V_min"
  dV/1 -> dV_big/1  "dV"
  derate/1 -> Warn_word_cat/6  "derate"
  Fan_Cmd/1 -> RT_fan/1  "Fan_Cmd"
  est_SOC_pack/1 -> RT_SOC/1  "SOC_pack"
  m_V_max_2/1 -> At_top/1  "V_max"
  m_Safety_OK/1 -> Safety_open/1  "Safety_OK"
  dV_big/1 -> Imbalance/1  "dV_big"
  At_top/1 -> Imbalance/2  "At_top"
  Safety_open/1 -> Lvl1/2, Aux_word_cat/17  "Safety_open"
  RT_SOC/1 -> SOC_low/1, SOC_crit/1  "RT_SOC"
  RT_fan/1 -> Fan_warn/1  "RT_fan"
  Aux_word_zero/1 -> Aux_word_cat/32, Aux_word_cat/31, Aux_word_cat/30, Aux_word_cat/29, Aux_word_cat/28, Aux_word_cat/27, Aux_word_cat/1, Aux_word_cat/26, Aux_word_cat/2, Aux_word_cat/25, Aux_word_cat/3, Aux_word_cat/24, Aux_word_cat/4, Aux_word_cat/23, Aux_word_cat/5, Aux_word_cat/22, Aux_word_cat/6, Aux_word_cat/20, Aux_word_cat/19, Aux_word_cat/9, Aux_word_cat/18, Aux_word_cat/10, Aux_word_cat/11, Aux_word_cat/16, Aux_word_cat/12, Aux_word_cat/15, Aux_word_cat/13, Aux_word_cat/14  "Aux_word_zero"
  m_T_max/1 -> OT_warn/1  "T_max"
  mode_Fault_PrechargeFail/1 -> Aux_word_cat/7  "Fault_PrechargeFail"
  mode_Fault_Weld/1 -> Aux_word_cat/8  "Fault_Weld"
  mode_mcu_timeout/1 -> Aux_word_cat/21  "mcu_timeout"
  Aux_word_cat/1 -> Aux_word/1  "Aux_word_cat"
  OT_warn/1 -> Warn_word_cat/3  "OT_warn"
  SOC_low/1 -> Warn_word_cat/4  "SOC_low"
  SOC_crit/1 -> Warn_word_cat/5  "SOC_crit"
  Imbalance/1 -> Warn_word_cat/7  "Imbalance"
  Fan_warn/1 -> Warn_word_cat/8  "Fan_warn"
  Warn_word_zero/1 -> Warn_word_cat/9, Warn_word_cat/32, Warn_word_cat/10, Warn_word_cat/31, Warn_word_cat/11, Warn_word_cat/30, Warn_word_cat/12, Warn_word_cat/29, Warn_word_cat/13, Warn_word_cat/28, Warn_word_cat/14, Warn_word_cat/27, Warn_word_cat/15, Warn_word_cat/26, Warn_word_cat/16, Warn_word_cat/25, Warn_word_cat/17, Warn_word_cat/24, Warn_word_cat/18, Warn_word_cat/23, Warn_word_cat/19, Warn_word_cat/22, Warn_word_cat/20, Warn_word_cat/21  "Warn_word_zero"
  prot_uv_warn/1 -> Warn_word_cat/1  "uv_warn"
  prot_ov_warn/1 -> Warn_word_cat/2  "ov_warn"
  Warn_word_cat/1 -> Warn_word/1  "Warn_word_cat"
  Aux_word/1 -> FW_or/2  "Aux_word"
  prot_latched/1 -> FW_or/1  "latched"
  FW_or/1 -> fw_Fault_Word/1, Lvl2_mask/1, Lvl3_mask/1  "Fault_Word"
  Warn_word/1 -> fw_Warning_Word/1, Warn_any/1  "Warning_Word"
  Warn_any/1 -> Lvl1/1  "Warn_any"
  Lvl2_mask/1 -> Lvl2/1  "Lvl2_mask"
  Lvl3_mask/1 -> Lvl3/1  "Lvl3_mask"
  Lvl1/1 -> L1_u8/1  "Lvl1"
  Lvl2/1 -> L2_u8/1  "Lvl2"
  Lvl3/1 -> L3_u8/1  "Lvl3"
  L1_u8/1 -> L1_w/1  "L1_u8"
  L2_u8/1 -> L2_w/1  "L2_u8"
  L3_u8/1 -> L3_w/1  "L3_u8"
  L1_w/1 -> Level_max/1  "L1_w"
  L2_w/1 -> Level_max/2  "L2_w"
  L3_w/1 -> Level_max/3  "L3_w"
  Level_max/1 -> fw_Fault_Level/1  "Fault_Level"

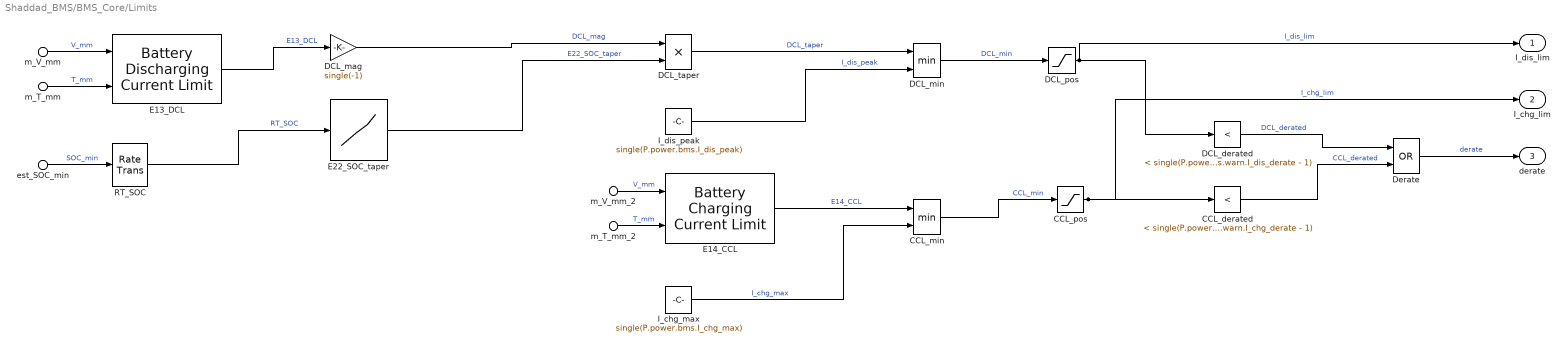
== system Shaddad_BMS/BMS_Core/Limits ==
  m_V_mm : Inport  PortName=m  Element=V_mm
  m_V_mm_2 : Inport  PortName=m  Element=V_mm
  m_T_mm : Inport  PortName=m  Element=T_mm
  m_T_mm_2 : Inport  PortName=m  Element=T_mm
  est_SOC_min : Inport  Port=2  PortName=est  Element=SOC_min
  CCL_derated : simulink/Logic and Bit Operations/Compare To Constant  relop=<  const=single(P.power.bms.warn.I_chg_derate - 1)  OutDataTypeStr=boolean
  CCL_min : MinMax  Inputs=2
  CCL_pos : Saturate  UpperLimit=inf  LowerLimit=0
  DCL_derated : simulink/Logic and Bit Operations/Compare To Constant  relop=<  const=single(P.power.bms.warn.I_dis_derate - 1)  OutDataTypeStr=boolean
  DCL_mag : Gain  Gain=single(-1)
  DCL_min : MinMax  Inputs=2
  DCL_pos : Saturate  UpperLimit=inf  LowerLimit=0
  DCL_taper : Product
  Derate : Logic  Operator=OR  AllPortsSameDT=off  OutDataTypeStr=boolean
  E13_DCL : BatteryCurrentManagement/Battery Discharging Current Limit  MinMaxFlag=on  CellUndervoltageLimit=single(P.power.bms.V_uv)  R0=single(P.power.bms.R0_limit)  T_vec=single(P.power.bms.dis.T_vec)  CurrentLimitCoolestCell=single(P.power.bms.dis.I_cool)  CurrentLimitHottestCell=single(P.power.bms.dis.I_hot)  DataType=Inherit: auto
      settings: LibrarySourceBlock=|
      | batt_sl_lib/Current Management/Battery Discharging
      | Current Limit
  E14_CCL : BatteryCurrentManagement/Battery Charging Current Limit  MinMaxFlag=on  CellOvervoltageLimit=single(P.power.bms.V_ov_warn)  R0=single(P.power.bms.R0_limit)  T_vec=single(P.power.bms.chg.T_vec)  CurrentLimitCoolestCell=single(P.power.bms.chg.I_cool)  CurrentLimitHottestCell=single(P.power.bms.chg.I_hot)  DataType=Inherit: auto
      settings: LibrarySourceBlock=|
      | batt_sl_lib/Current Management/Battery Charging
      | Current Limit
  E22_SOC_taper : Lookup_n-D  NumberOfTableDimensions=1  BreakpointsForDimension1=single(P.power.bms.soc_taper.bp)  Table=single(P.power.bms.soc_taper.k)  InterpMethod=Flat  ExtrapMethod=Clip  InternalRulePriority=Speed  RndMeth=Simplest
  I_chg_max : Constant  Value=single(P.power.bms.I_chg_max)  OutDataTypeStr=single  SampleTime=Ts.bms_fast
  I_dis_peak : Constant  Value=single(P.power.bms.I_dis_peak)  OutDataTypeStr=single  SampleTime=Ts.bms_fast
  RT_SOC : RateTransition  InitialCondition=single(min(P.power.bms.est.SOC_init))  OutPortSampleTime=Ts.bms_fast
  I_dis_lim : Outport
  I_chg_lim : Outport  Port=2
  derate : Outport  Port=3
  wires:
  m_V_mm/1 -> E13_DCL/1  "V_mm"
  m_T_mm/1 -> E13_DCL/2  "T_mm"
  est_SOC_min/1 -> RT_SOC/1  "SOC_min"
  RT_SOC/1 -> E22_SOC_taper/1  "RT_SOC"
  E13_DCL/1 -> DCL_mag/1  "E13_DCL"
  DCL_mag/1 -> DCL_taper/1  "DCL_mag"
  E22_SOC_taper/1 -> DCL_taper/2  "E22_SOC_taper"
  m_V_mm_2/1 -> E14_CCL/1  "V_mm"
  m_T_mm_2/1 -> E14_CCL/2  "T_mm"
  DCL_taper/1 -> DCL_min/1  "DCL_taper"
  I_dis_peak/1 -> DCL_min/2  "I_dis_peak"
  I_chg_max/1 -> CCL_min/2  "I_chg_max"
  E14_CCL/1 -> CCL_min/1  "E14_CCL"
  DCL_min/1 -> DCL_pos/1  "DCL_min"
  CCL_min/1 -> CCL_pos/1  "CCL_min"
  DCL_pos/1 -> DCL_derated/1, I_dis_lim/1  "I_dis_lim"
  CCL_pos/1 -> I_chg_lim/1, CCL_derated/1  "I_chg_lim"
  DCL_derated/1 -> Derate/1  "DCL_derated"
  CCL_derated/1 -> Derate/2  "CCL_derated"
  Derate/1 -> derate/1  "derate"

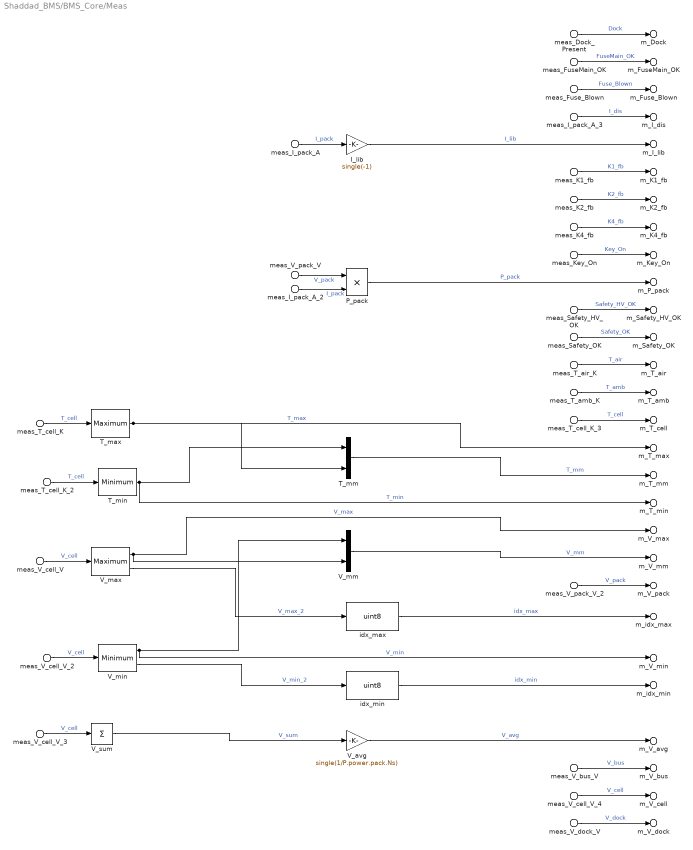
== system Shaddad_BMS/BMS_Core/Meas ==
  meas_V_cell_V : Inport  PortName=meas  Element=V_cell_V
  meas_V_cell_V_2 : Inport  PortName=meas  Element=V_cell_V
  meas_V_cell_V_3 : Inport  PortName=meas  Element=V_cell_V
  meas_V_cell_V_4 : Inport  PortName=meas  Element=V_cell_V
  meas_T_cell_K : Inport  PortName=meas  Element=T_cell_K
  meas_T_cell_K_2 : Inport  PortName=meas  Element=T_cell_K
  meas_T_cell_K_3 : Inport  PortName=meas  Element=T_cell_K
  meas_I_pack_A : Inport  PortName=meas  Element=I_pack_A
  meas_I_pack_A_2 : Inport  PortName=meas  Element=I_pack_A
  meas_I_pack_A_3 : Inport  PortName=meas  Element=I_pack_A
  meas_V_pack_V : Inport  PortName=meas  Element=V_pack_V
  meas_V_pack_V_2 : Inport  PortName=meas  Element=V_pack_V
  meas_V_bus_V : Inport  PortName=meas  Element=V_bus_V
  meas_V_dock_V : Inport  PortName=meas  Element=V_dock_V
  meas_T_amb_K : Inport  PortName=meas  Element=T_amb_K
  meas_T_air_K : Inport  PortName=meas  Element=T_air_K
  meas_K1_fb : Inport  PortName=meas  Element=K1_fb
  meas_K2_fb : Inport  PortName=meas  Element=K2_fb
  meas_K4_fb : Inport  PortName=meas  Element=K4_fb
  meas_Dock_Present : Inport  PortName=meas  Element=Dock_Present
  meas_Safety_OK : Inport  PortName=meas  Element=Safety_OK
  meas_Safety_HV_OK : Inport  PortName=meas  Element=Safety_HV_OK
  meas_Key_On : Inport  PortName=meas  Element=Key_On
  meas_FuseMain_OK : Inport  PortName=meas  Element=FuseMain_OK
  meas_Fuse_Blown : Inport  PortName=meas  Element=Fuse_Blown
  I_lib : Gain  Gain=single(-1)
  P_pack : Product
  T_max : dspstat3/Maximum  operation=maximum  fcn=Value  indexBase=One  operateOver=Each column  Dimension=1  InputProcessing=Columns as channels (frame based)  reset=None  roiEnable=off  roiType=Rectangles  roiPortion=Entire ROI  roiOutput=Individual statistics for each ROI  roiFlag=off  roundingMode=Floor  overflowMode=off  accumDataTypeStr=Inherit: Same as product output  accumLastDataTypeStr=Inherit: Same as product output
  T_min : dspstat3/Minimum  operation=minimum  fcn=Value  indexBase=One  operateOver=Each column  Dimension=1  InputProcessing=Columns as channels (frame based)  reset=None  roiEnable=off  roiType=Rectangles  roiPortion=Entire ROI  roiOutput=Individual statistics for each ROI  roiFlag=off  roundingMode=Floor  overflowMode=off
  T_mm : Mux  Inputs=2
  V_avg : Gain  Gain=single(1/P.power.pack.Ns)
  V_max : dspstat3/Maximum  operation=maximum  fcn=Value and Index  indexBase=One  operateOver=Each column  Dimension=1  InputProcessing=Columns as channels (frame based)  reset=None  roiEnable=off  roiType=Rectangles  roiPortion=Entire ROI  roiOutput=Individual statistics for each ROI  roiFlag=off  roundingMode=Floor  overflowMode=off  accumDataTypeStr=Inherit: Same as product output  accumLastDataTypeStr=Inherit: Same as product output
  V_min : dspstat3/Minimum  operation=minimum  fcn=Value and Index  indexBase=One  operateOver=Each column  Dimension=1  InputProcessing=Columns as channels (frame based)  reset=None  roiEnable=off  roiType=Rectangles  roiPortion=Entire ROI  roiOutput=Individual statistics for each ROI  roiFlag=off  roundingMode=Floor  overflowMode=off
  V_mm : Mux  Inputs=2
  V_sum : Sum  Inputs=+
  idx_max : DataTypeConversion  OutDataTypeStr=uint8  RndMeth=Nearest
  idx_min : DataTypeConversion  OutDataTypeStr=uint8  RndMeth=Nearest
  m_V_cell : Outport  PortName=m  Element=V_cell
  m_T_cell : Outport  PortName=m  Element=T_cell
  m_I_dis : Outport  PortName=m  Element=I_dis
  m_I_lib : Outport  PortName=m  Element=I_lib
  m_V_pack : Outport  PortName=m  Element=V_pack
  m_V_bus : Outport  PortName=m  Element=V_bus
  m_V_dock : Outport  PortName=m  Element=V_dock
  m_T_amb : Outport  PortName=m  Element=T_amb
  m_T_air : Outport  PortName=m  Element=T_air
  m_V_min : Outport  PortName=m  Element=V_min
  m_V_max : Outport  PortName=m  Element=V_max
  m_V_avg : Outport  PortName=m  Element=V_avg
  m_idx_min : Outport  PortName=m  Element=idx_min
  m_idx_max : Outport  PortName=m  Element=idx_max
  m_T_min : Outport  PortName=m  Element=T_min
  m_T_max : Outport  PortName=m  Element=T_max
  m_V_mm : Outport  PortName=m  Element=V_mm
  m_T_mm : Outport  PortName=m  Element=T_mm
  m_P_pack : Outport  PortName=m  Element=P_pack
  m_K1_fb : Outport  PortName=m  Element=K1_fb
  m_K2_fb : Outport  PortName=m  Element=K2_fb
  m_K4_fb : Outport  PortName=m  Element=K4_fb
  m_Dock : Outport  PortName=m  Element=Dock
  m_Safety_OK : Outport  PortName=m  Element=Safety_OK
  m_Safety_HV_OK : Outport  PortName=m  Element=Safety_HV_OK
  m_Key_On : Outport  PortName=m  Element=Key_On
  m_FuseMain_OK : Outport  PortName=m  Element=FuseMain_OK
  m_Fuse_Blown : Outport  PortName=m  Element=Fuse_Blown
  wires:
  meas_T_cell_K/1 -> T_max/1  "T_cell"
  meas_V_cell_V/1 -> V_max/1  "V_cell"
  meas_V_cell_V_3/1 -> V_sum/1  "V_cell"
  meas_T_cell_K_2/1 -> T_min/1  "T_cell"
  meas_V_cell_V_2/1 -> V_min/1  "V_cell"
  V_sum/1 -> V_avg/1  "V_sum"
  T_max/1 -> T_mm/2, m_T_max/1  "T_max"
  V_max/1 -> m_V_max/1, V_mm/2  "V_max"
  V_max/2 -> idx_max/1  "V_max_2"
  T_min/1 -> T_mm/1, m_T_min/1  "T_min"
  V_min/1 -> V_mm/1, m_V_min/1  "V_min"
  V_min/2 -> idx_min/1  "V_min_2"
  meas_I_pack_A/1 -> I_lib/1  "I_pack"
  meas_V_pack_V/1 -> P_pack/1  "V_pack"
  meas_I_pack_A_2/1 -> P_pack/2  "I_pack"
  T_mm/1 -> m_T_mm/1  "T_mm"
  V_mm/1 -> m_V_mm/1  "V_mm"
  I_lib/1 -> m_I_lib/1  "I_lib"
  P_pack/1 -> m_P_pack/1  "P_pack"
  V_avg/1 -> m_V_avg/1  "V_avg"
  idx_max/1 -> m_idx_max/1  "idx_max"
  idx_min/1 -> m_idx_min/1  "idx_min"
  meas_Dock_Present/1 -> m_Dock/1  "Dock"
  meas_FuseMain_OK/1 -> m_FuseMain_OK/1  "FuseMain_OK"
  meas_Fuse_Blown/1 -> m_Fuse_Blown/1  "Fuse_Blown"
  meas_I_pack_A_3/1 -> m_I_dis/1  "I_dis"
  meas_K1_fb/1 -> m_K1_fb/1  "K1_fb"
  meas_K2_fb/1 -> m_K2_fb/1  "K2_fb"
  meas_K4_fb/1 -> m_K4_fb/1  "K4_fb"
  meas_Key_On/1 -> m_Key_On/1  "Key_On"
  meas_Safety_HV_OK/1 -> m_Safety_HV_OK/1  "Safety_HV_OK"
  meas_Safety_OK/1 -> m_Safety_OK/1  "Safety_OK"
  meas_T_air_K/1 -> m_T_air/1  "T_air"
  meas_T_amb_K/1 -> m_T_amb/1  "T_amb"
  meas_T_cell_K_3/1 -> m_T_cell/1  "T_cell"
  meas_V_pack_V_2/1 -> m_V_pack/1  "V_pack"
  meas_V_bus_V/1 -> m_V_bus/1  "V_bus"
  meas_V_cell_V_4/1 -> m_V_cell/1  "V_cell"
  meas_V_dock_V/1 -> m_V_dock/1  "V_dock"
